simulink library "PacketizedNetworkLib"  (R2025b)
settings: Solver=VariableStepAuto  StartTime=0.0  StopTime=10.0  RelTol=1e-3
values from neighbouring files (symbols this model uses):
  dfeRef = [0.707106781187 -0.707106781187 0.707106781187 0.707106781187 -0.707106781187 0.707106781187 0.707106781187 0.707106781187 0.707106781187 0.707106781187 -0.707106781187 0.707106781187 ... (500 elements, 500x1)]    [networkParams.mat]
  L3payload = [0 0 0 1 0 0 0 0 1 1 1 0 ... (1040 elements, 1040x1)]    [networkParams.mat]
  ppdu_bb = [0 0 1 1 0 0 0 0 1 1 0 0 ... (2280 elements, 2280x1)]    [networkParams.mat]
  Ts = 1e-07    [networkParams.mat]
undefined symbols (not defined in the file or in its folder): AckDestAddre, DestAddre, dfilt, High, lambda, NodeAddre, pseed
libraries: $bdroot x19, hdlsllib x5, dspsigops x5, dspswit3 x3, simulink x3, dspindex x3, commdigbbndpm3 x2, simulink_extras x2, commfilt2 x2, commchan3 x1, dspmathops x1, dsparch4 x1
(part 1 of 3)
settings Model: Creator=The MathWorks, Inc.  LastModifiedBy=The MathWorks, Inc.
settings SolverCC: AlgebraicLoopSolver=TrustRegion
settings DataIOCC: ReturnWorkspaceOutputs=off
settings OptimizationCC: ReuseModelBlockBuffer=off
settings DebuggingCC: UnconnectedInputMsg=warning  UnconnectedOutputMsg=warning  UnconnectedLineMsg=warning  ArithmeticOperatorsInVariantConditions=warning
settings ModelReferenceCC: EnableRefExpFcnMdlSchedulingChecks=on
settings SFSimCC: SimUseLocalCustomCode=off  CustomCodeUndefinedFunction=UseInterfaceOnly
settings RTWCC: RTWUseLocalCustomCode=off  GPUComputeCapability=3.5

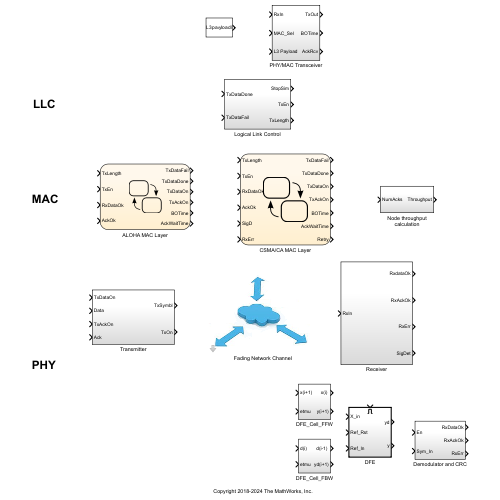
[thumbnail: Simulink's stored preview of the top-level diagram]
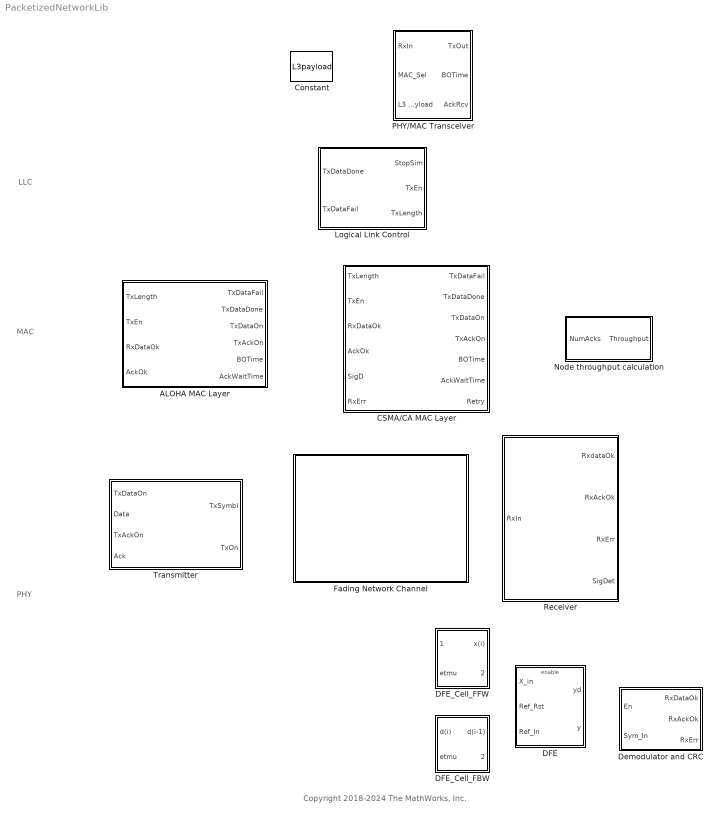
== system PacketizedNetworkLib ==
  note: PHY
  note: MAC
  note: LLC
  note: Copyright 2018-2024 The MathWorks, Inc.
  ALOHA MAC Layer : Stateflow chart  TreatAsAtomicUnit=on
  CSMA/CA MAC Layer : Stateflow chart  TreatAsAtomicUnit=on
  Constant : Constant  Value=L3payload
  DFE : Subsystem
  DFE_Cell_FBW : Subsystem
  DFE_Cell_FFW : Subsystem
  Demodulator and CRC : Subsystem
  Fading Network Channel : Subsystem  mask(Radio Network){MDSN12=0.000005/Ts, SNRN12=25, MDSN23=0.000005/Ts, SNRN23=25, MDSN31=0.000005/Ts, SNRN31=25}
      mask prompts: MDSN12 "Maximum Doppler Shift (Hz)"; SNRN12 "SNR of AWGN (Eb/No)"; MDSN23 "Maximum Doppler Shift (Hz)"; SNRN23 "SNR of AWGN (Eb/No)"; MDSN31 "Maximum Doppler Shift (Hz)"; SNRN31 "SNR of AWGN (Eb/No)"
      mask help: This model presents a radio network with Rayleigh fading channel between the transceiver nades.
      mask DialogControl ParameterGroupVar Prompt: Parameters for Channels
      mask DialogControl Container3 Prompt: Channel between Node 1 and Node 2
      mask DialogControl Container4 Prompt: Node 2 and Node 3
      mask DialogControl Container5 Prompt: Node 3 and Node 1
      mask Display: image('NetworkChannel.png');
  Logical Link Control : Subsystem
  Node throughput calculation : Subsystem
  PHY/MAC Transceiver : Subsystem
  Receiver : Subsystem
  Transmitter : Subsystem  Tag=safddsaf  Description=afsd as

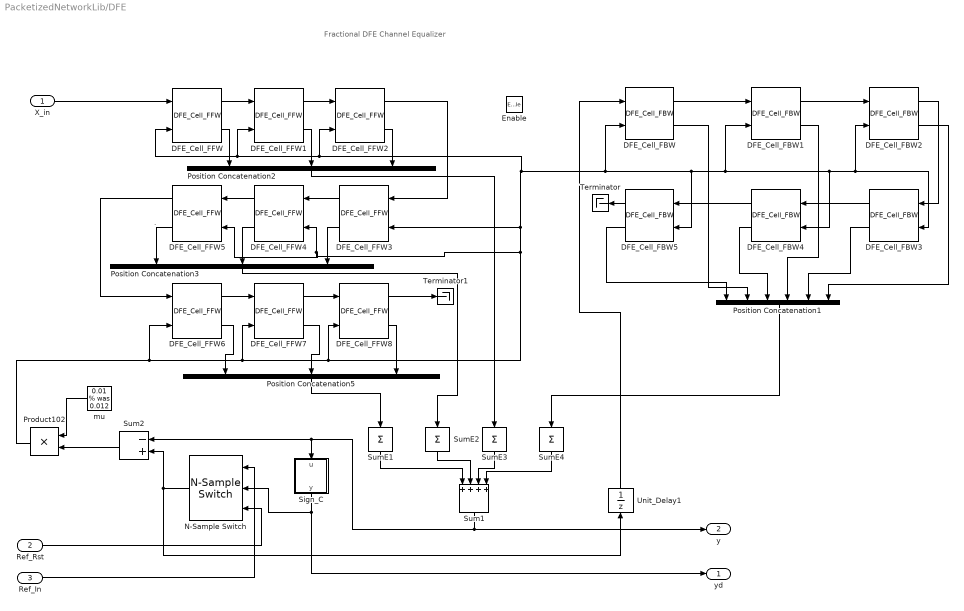
== system PacketizedNetworkLib/DFE ==
  note: .
  note: Fractional DFE Channel Equalizer
  X_in : Inport
  "Ref_Rst " : Inport  Port=2
  Ref_In : Inport  Port=3
  Enable : EnablePort
  DFE_Cell_FBW{,1..5} (6 alike) : $bdroot/DFE_Cell_FBW  SystemSampleTime=-1  VariantActivationTime=update diagram  EmptyChoice=off  PassThrough=off  PassThroughVariantControl=(default)  EmptyChoiceVariantControl=(default)  AllowFlexibleInterface=on  Latency=0  AutoFrameSizeCalculation=off
  DFE_Cell_FFW{,1..8} (9 alike) : $bdroot/DFE_Cell_FFW  SystemSampleTime=-1  VariantActivationTime=update diagram  EmptyChoice=off  PassThrough=off  PassThroughVariantControl=(default)  EmptyChoiceVariantControl=(default)  AllowFlexibleInterface=on  Latency=0  AutoFrameSizeCalculation=off
  N-Sample Switch : dspswit3/N-Sample Switch  N=152  reset=on  TriggerType=Rising edge  Ts=-1
  Position Concatenation1 : Concatenate  NumInputs=6  ConcatenateDimension=6
  Position Concatenation2 : Concatenate  NumInputs=3  ConcatenateDimension=3
  Position Concatenation3 : Concatenate  NumInputs=3  ConcatenateDimension=3
  Position Concatenation5 : Concatenate  NumInputs=3  ConcatenateDimension=3
  Product102 : Product  InputSameDT=on  RndMeth=Zero  SaturateOnIntegerOverflow=on  OutDataTypeStr=Inherit: Same as first input
  "Sign_C " : MATLAB Function  TreatAsAtomicUnit=on
  Sum1 : Sum  Inputs=++++  InputSameDT=on  SaturateOnIntegerOverflow=on  OutDataTypeStr=Inherit: Same as first input
  Sum2 : Sum  Inputs=-+  InputSameDT=on  SaturateOnIntegerOverflow=on  OutDataTypeStr=Inherit: Same as first input
  SumE{1..4} (4 alike) : Sum  Inputs=+
  Terminator : Terminator
  Terminator1 : Terminator
  "Unit_Delay1 " : UnitDelay  SampleTime=-1  HasFrameUpgradeWarning=on
  mu : Constant  Value="0.01  % was 0.012"  SampleTime=-1
  yd : Outport  VectorParamsAs1DForOutWhenUnconnected=off
  y : Outport  Port=2  VectorParamsAs1DForOutWhenUnconnected=off
  wires:
  DFE_Cell_FFW4/1 -> DFE_Cell_FFW5/1
  DFE_Cell_FFW3/2 -> Position Concatenation3/3
  Position Concatenation2/1 -> SumE3/1
  Position Concatenation3/1 -> SumE2/1
  DFE_Cell_FBW3/1 -> DFE_Cell_FBW4/1
  DFE_Cell_FFW7/2 -> Position Concatenation5/2
  DFE_Cell_FBW/1 -> DFE_Cell_FBW1/1
  DFE_Cell_FFW5/2 -> Position Concatenation3/1
  "Unit_Delay1 "/1 -> DFE_Cell_FBW/1
  DFE_Cell_FFW6/2 -> Position Concatenation5/1
  "Sign_C "/1(y) -> yd/1, N-Sample Switch/2
  DFE_Cell_FFW8/2 -> Position Concatenation5/3
  SumE2/1 -> Sum1/2
  DFE_Cell_FFW2/2 -> Position Concatenation2/3
  DFE_Cell_FFW8/1 -> Terminator1/1
  DFE_Cell_FFW5/1 -> DFE_Cell_FFW6/1
  Sum1/1 -> y/1, "Sign_C "/1(u), Sum2/1
  DFE_Cell_FFW1/2 -> Position Concatenation2/2
  DFE_Cell_FBW/2 -> Position Concatenation1/2
  DFE_Cell_FFW/2 -> Position Concatenation2/1
  SumE1/1 -> Sum1/1
  DFE_Cell_FFW3/1 -> DFE_Cell_FFW4/1
  DFE_Cell_FFW4/2 -> Position Concatenation3/2
  DFE_Cell_FBW5/1 -> Terminator/1
  Sum2/1 -> Product102/2
  DFE_Cell_FBW2/1 -> DFE_Cell_FBW3/1
  Product102/1 -> DFE_Cell_FFW6/2, DFE_Cell_FFW7/2, DFE_Cell_FFW8/2, DFE_Cell_FFW5/2, DFE_Cell_FFW4/2, DFE_Cell_FFW3/2, DFE_Cell_FFW2/2, DFE_Cell_FFW1/2, DFE_Cell_FFW/2, DFE_Cell_FBW/2, DFE_Cell_FBW5/2, DFE_Cell_FBW1/2, DFE_Cell_FBW4/2, DFE_Cell_FBW3/2, DFE_Cell_FBW2/2
  SumE3/1 -> Sum1/3
  mu/1 -> Product102/1
  N-Sample Switch/1 -> "Unit_Delay1 "/1, Sum2/2
  Position Concatenation1/1 -> SumE4/1
  DFE_Cell_FFW2/1 -> DFE_Cell_FFW3/1
  DFE_Cell_FFW1/1 -> DFE_Cell_FFW2/1
  DFE_Cell_FBW1/2 -> Position Concatenation1/4
  DFE_Cell_FBW3/2 -> Position Concatenation1/5
  DFE_Cell_FBW4/2 -> Position Concatenation1/3
  DFE_Cell_FBW4/1 -> DFE_Cell_FBW5/1
  DFE_Cell_FBW5/2 -> Position Concatenation1/1
  DFE_Cell_FBW1/1 -> DFE_Cell_FBW2/1
  SumE4/1 -> Sum1/4
  DFE_Cell_FFW/1 -> DFE_Cell_FFW1/1
  Position Concatenation5/1 -> SumE1/1
  DFE_Cell_FBW2/2 -> Position Concatenation1/6
  DFE_Cell_FFW6/1 -> DFE_Cell_FFW7/1
  DFE_Cell_FFW7/1 -> DFE_Cell_FFW8/1
  Ref_In/1 -> N-Sample Switch/1
  X_in/1 -> DFE_Cell_FFW/1
  "Ref_Rst "/1 -> N-Sample Switch/3

== system PacketizedNetworkLib/DFE_Cell_FBW ==
  note: w(i+1)
  note: The Basic Cell of the Feedbackward Part of DFE Equalizer
      |
      | yd(i+1)= w(i+1).*d(i);
      | w(i+1)=w(i)+ m*D* w(i)=w(i)+etmu*conj(x(i));
      |
      | Note: All variables here are scalars
  note: w(i)
  d(i) : Inport
  etmu : Inport  Port=2
  " Unit_Delay1" : UnitDelay  SampleTime=-1  HasFrameUpgradeWarning=on
  " Unit_Delay2" : UnitDelay  SampleTime=-1  HasFrameUpgradeWarning=on
  Math Function : Math  Operator=conj  SignedPower=on
  Product1 : Product  InputSameDT=on  RndMeth=Zero  SaturateOnIntegerOverflow=on  OutDataTypeStr=Inherit: Same as first input
  Product2 : Product  InputSameDT=on  RndMeth=Zero  SaturateOnIntegerOverflow=on  OutDataTypeStr=Inherit: Same as first input
  Sum : Sum  InputSameDT=on  SaturateOnIntegerOverflow=on  OutDataTypeStr=Inherit: Same as first input
  "Unit_Delay1 " : UnitDelay  SampleTime=-1  HasFrameUpgradeWarning=on
  "d(i-1) " : Outport  VectorParamsAs1DForOutWhenUnconnected=off
  yd(i+1) : Outport  Port=2  VectorParamsAs1DForOutWhenUnconnected=off
  wires:
  Product2/1 -> Sum/2
  Product1/1 -> yd(i+1)/1
  Sum/1 -> Product1/1, " Unit_Delay2"/1
  " Unit_Delay2"/1 -> Sum/1
  "Unit_Delay1 "/1 -> Math Function/1, "d(i-1) "/1
  etmu/1 -> " Unit_Delay1"/1
  d(i)/1 -> Product1/2, "Unit_Delay1 "/1
  Math Function/1 -> Product2/2
  " Unit_Delay1"/1 -> Product2/1

== system PacketizedNetworkLib/DFE_Cell_FFW ==
  note: w(i)
  note: The Basic Cell of the Feedforward Part of DFE Equalizer
      |
      | y(i+1)= ElimentSum (w(i+1).*x(i+1));
      | w(i+1)=w(i)+ m*D* w(i)=w(i)+etmu*conj(x(i));
      |
      | Note: y(+1) and etmu is a scalar, and x(i), w(i) are 2x1 vector. "2" is the decimation factor 2
  note: w(i+1)
  x(i+1) : Inport
  etmu : Inport  Port=2
  " Unit_Delay1" : UnitDelay  SampleTime=-1  HasFrameUpgradeWarning=on
  " Unit_Delay2" : UnitDelay  SampleTime=-1  HasFrameUpgradeWarning=on
  Math Function : Math  Operator=conj  SignedPower=on
  Product1 : Product  InputSameDT=on  RndMeth=Zero  SaturateOnIntegerOverflow=on  OutDataTypeStr=Inherit: Same as first input
  Product2 : Product  InputSameDT=on  RndMeth=Zero  SaturateOnIntegerOverflow=on  OutDataTypeStr=Inherit: Same as first input
  Sum : Sum  InputSameDT=on  SaturateOnIntegerOverflow=on  OutDataTypeStr=Inherit: Same as first input
  Sum of Elements : Sum  Inputs=+
  "Unit_Delay1 " : UnitDelay  SampleTime=-1  HasFrameUpgradeWarning=on
  "x(i) " : Outport  VectorParamsAs1DForOutWhenUnconnected=off
  y(i+1) : Outport  Port=2  VectorParamsAs1DForOutWhenUnconnected=off
  wires:
  " Unit_Delay1"/1 -> Product2/1
  Sum/1 -> " Unit_Delay2"/1, Product1/1
  Sum of Elements/1 -> y(i+1)/1
  Math Function/1 -> Product2/2
  x(i+1)/1 -> "Unit_Delay1 "/1, Product1/2
  etmu/1 -> " Unit_Delay1"/1
  "Unit_Delay1 "/1 -> "x(i) "/1, Math Function/1
  " Unit_Delay2"/1 -> Sum/1
  Product1/1 -> Sum of Elements/1
  Product2/1 -> Sum/2

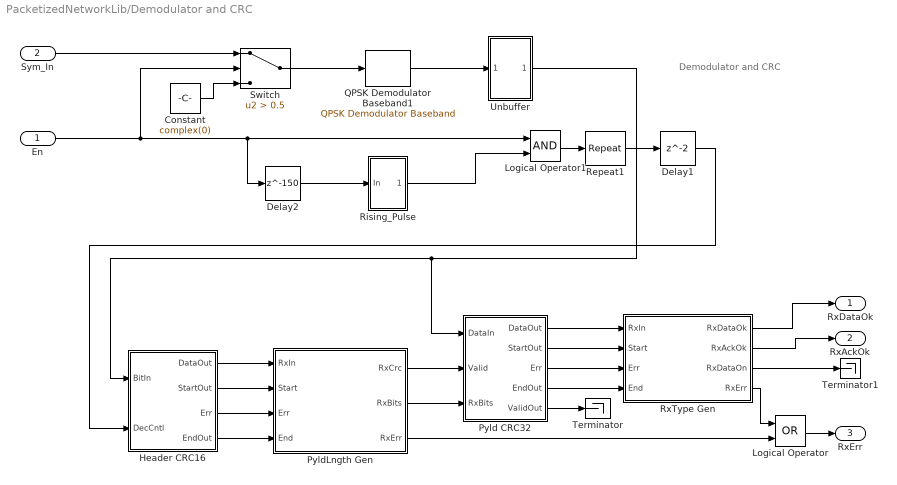
== system PacketizedNetworkLib/Demodulator and CRC ==
  note: Demodulator and CRC
  En : Inport
  Sym_In : Inport  Port=2
  " QPSK Demodulator Baseband1" : commdigbbndpm3/QPSK Demodulator Baseband  OutType=Bit  DecType=Hard decision  VarSource=Dialog  Variance=1  Dec=Gray  Ph=pi/4  outDtype1=Inherit via internal rule  outDtype2=Inherit via internal rule  derotateFactorWordLen=16  derotateFactorDataTypeStr=Inherit: Same word length as input  derotateFactorLastDataTypeStr=Inherit: Same word length as input
  Constant : Constant  Value=complex(0)  OutDataTypeStr=fixdt(1,16,14)  SampleTime=-1
  Delay1 : Delay
  Delay2 : Delay  DelayLength=150
  "Header CRC16 " : Subsystem
  Logical Operator : Logic  Operator=OR  AllPortsSameDT=off  OutDataTypeStr=boolean
  Logical Operator1 : Logic  AllPortsSameDT=off  OutDataTypeStr=boolean
  Pyld CRC32 : Subsystem
  PyldLngth Gen : Stateflow chart  TreatAsAtomicUnit=on
  Repeat1 : dspsigops/Repeat  FactorSource=Dialog parameter  N=2  Nmax=16  RateOptions=Allow multirate processing  ic=0  mode=Unused parameter value
  Rising_Pulse : Subsystem
  RxType Gen : Stateflow chart  TreatAsAtomicUnit=on
  Switch : Switch  Criteria=u2 > Threshold  Threshold=0.5  SaturateOnIntegerOverflow=off  InputSameDT=off
  Terminator : Terminator
  Terminator1 : Terminator
  Unbuffer : Subsystem
  RxDataOk : Outport  VectorParamsAs1DForOutWhenUnconnected=off
  RxAckOk : Outport  Port=2  VectorParamsAs1DForOutWhenUnconnected=off
  RxErr : Outport  Port=3  VectorParamsAs1DForOutWhenUnconnected=off
  wires:
  Pyld CRC32/1(DataOut) -> RxType Gen/1(RxIn)
  Switch/1 -> " QPSK Demodulator Baseband1"/1
  Constant/1 -> Switch/3
  Delay2/1 -> Rising_Pulse/1(In)
  Sym_In/1 -> Switch/1
  "Header CRC16 "/2(StartOut) -> PyldLngth Gen/2(Start)
  "Header CRC16 "/4(EndOut) -> PyldLngth Gen/4(End)
  "Header CRC16 "/3(Err) -> PyldLngth Gen/3(Err)
  PyldLngth Gen/1(RxCrc) -> Pyld CRC32/2(Valid)
  Rising_Pulse/1(Out1) -> Logical Operator1/2
  Unbuffer/1(Out1) -> Pyld CRC32/1(DataIn), "Header CRC16 "/1(BitIn)
  Pyld CRC32/2(StartOut) -> RxType Gen/2(Start)
  Pyld CRC32/3(Err) -> RxType Gen/3(Err)
  Pyld CRC32/4(EndOut) -> RxType Gen/4(End)
  RxType Gen/1(RxDataOk) -> RxDataOk/1
  RxType Gen/2(RxAckOk) -> RxAckOk/1
  En/1 -> Switch/2, Logical Operator1/1, Delay2/1
  " QPSK Demodulator Baseband1"/1 -> Unbuffer/1(In1)
  "Header CRC16 "/1(DataOut) -> PyldLngth Gen/1(RxIn)
  Pyld CRC32/5(ValidOut) -> Terminator/1
  PyldLngth Gen/3(RxErr) -> Logical Operator/2
  RxType Gen/4(RxErr) -> Logical Operator/1
  Logical Operator/1 -> RxErr/1
  Logical Operator1/1 -> Repeat1/1
  RxType Gen/3(RxDataOn) -> Terminator1/1
  PyldLngth Gen/2(RxBits) -> Pyld CRC32/3(RxBits)
  Repeat1/1 -> Delay1/1
  Delay1/1 -> "Header CRC16 "/2(DecCntl)

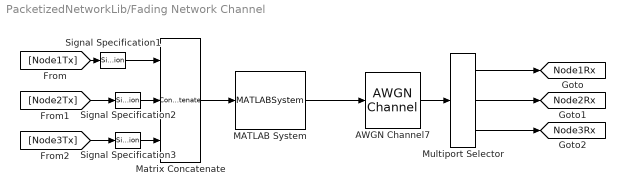
== system PacketizedNetworkLib/Fading Network Channel ==
  AWGN Channel7 : commchan3/AWGN Channel  LegacyMode=off  NoiseMethod="Signal to noise ratio  (Eb/No)"  noiseMode="Signal to noise ratio  (SNR)"  EbNo=[SNRN12, SNRN23, SNRN31]  EsNo=10  SNR=10  BitsPerSymbol=2  SignalPower=0.1634  SpecifySymbolPeriod=off  SamplesPerSymbol=1  SymbolPeriod=Ts  VarianceSource=Parameter  Variance=1  RandomStream=mt19937ar with seed  Seed=67  SimulateUsing=Code generation
  MATLAB System : MATLABSystem  System=NetworkChannel  SampleRateSource=Input port  SampleRate=[ 1e3, 2e3, 3e3 ]  PathDelays={[0 0.3*Ts], [0 0.3*Ts]; [0 0.3*Ts], [0 0.3*Ts]; [0 0.3*Ts], [0 0.3*Ts]}  AveragePathGains={[0 -6],[0 -6]; [0 -6],[0 -6]; [0 -6],[0 -6]}  MaximumDopplerShift=[MDSN12, MDSN31; MDSN23, MDSN12; MDSN31, MDSN23]  SimulateUsing=Code generation
      mask Type: NetworkChannel
  Matrix Concatenate : Concatenate  NumInputs=3  Mode=Multidimensional array  ConcatenateDimension=2
  Multiport Selector : dspindex/Multiport Selector  rowsOrCols=Columns  idxCellArray=num2cell(1:3)  idxErrMode=Clip Index
  Signal Specification1 : SignalSpecification  Dimensions=1
  Signal Specification2 : SignalSpecification  Dimensions=1
  Signal Specification3 : SignalSpecification  Dimensions=1
  tag scope: Node1Rx=global, Node2Rx=global, Node3Rx=global
  wires:
  [Node1Tx] -> Signal Specification1/1
  [Node2Tx] -> Signal Specification2/1
  [Node3Tx] -> Signal Specification3/1
  Matrix Concatenate/1 -> MATLAB System/1
  Signal Specification1/1 -> Matrix Concatenate/1
  Signal Specification2/1 -> Matrix Concatenate/2
  Signal Specification3/1 -> Matrix Concatenate/3
  Multiport Selector/1 -> [Node1Rx]
  Multiport Selector/2 -> [Node2Rx]
  Multiport Selector/3 -> [Node3Rx]
  AWGN Channel7/1 -> Multiport Selector/1
  MATLAB System/1 -> AWGN Channel7/1

== system PacketizedNetworkLib/Logical Link Control ==
  TxDataDone : Inport
  TxDataFail : Inport  Port=2
  Exponential Random Variable : Subsystem
  Logical Link Control : Stateflow chart  TreatAsAtomicUnit=on
  Terminator : Terminator
  Terminator1 : Terminator
  StopSim : Outport  VectorParamsAs1DForOutWhenUnconnected=off
  TxEn : Outport  Port=2  VectorParamsAs1DForOutWhenUnconnected=off
  TxLength : Outport  Port=3  VectorParamsAs1DForOutWhenUnconnected=off
  wires:
  Logical Link Control/2(TxEn) -> TxEn/1
  TxDataDone/1 -> Logical Link Control/1(TxDataDone)
  Logical Link Control/1(StopSim) -> StopSim/1
  Logical Link Control/5(TxMore) -> Terminator1/1
  TxDataFail/1 -> Logical Link Control/2(TxDataFail)
  Logical Link Control/4(TxWaitTime) -> Terminator/1
  Logical Link Control/3(TxLength) -> TxLength/1
  Exponential Random Variable/1(Out1) -> Logical Link Control/3(TxWaitUnits)

== system PacketizedNetworkLib/Node throughput calculation ==
  NumAcks : Inport
  Clock : Clock
  Cumulative Sum2 : dspmathops/Cumulative Sum  dim=Channels (running sum)  InputProcessing=Columns as channels (frame based)  reset_popup=None  roundingMode=Floor  overflowMode=off  outputDataTypeStr=Inherit: Same as accumulator  outputMin=[]  outputMax=[]  outputLastDataTypeStr=Inherit: Same as accumulator
  Data Type Conversion2 : DataTypeConversion  OutDataTypeStr=uint8  SaturateOnIntegerOverflow=off  RndMeth=Floor
  Data packet airtime : Constant  Value=(50+254+16+16+4+2+2+8+8+8+32+1040+32)/20e6
  Divide2 : Product  Inputs=*/
  Product2 : Product
  Throughput : Outport  VectorParamsAs1DForOutWhenUnconnected=off
  wires:
  Data packet airtime/1 -> Product2/2
  Cumulative Sum2/1 -> Product2/1
  Data Type Conversion2/1 -> Cumulative Sum2/1
  Product2/1 -> Divide2/1
  Divide2/1 -> Throughput/1
  Clock/1 -> Divide2/2
  NumAcks/1 -> Data Type Conversion2/1

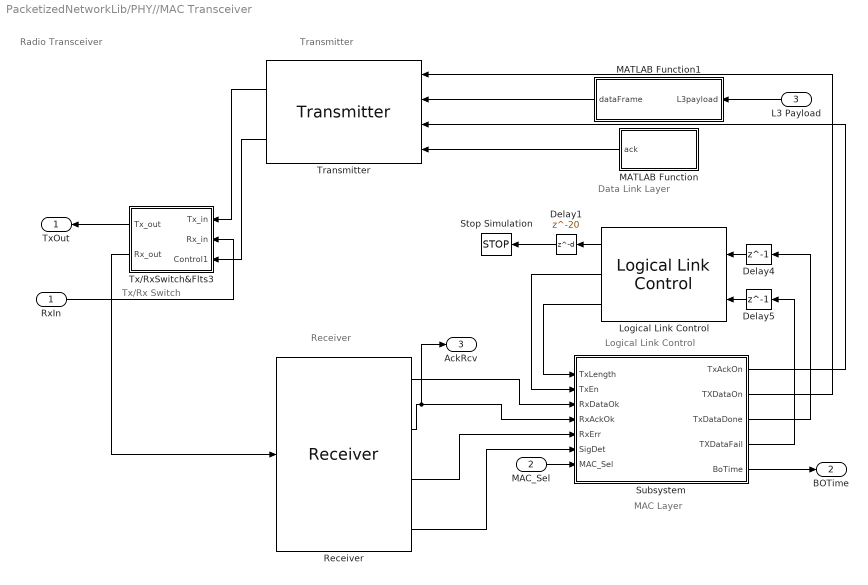
== system PacketizedNetworkLib/PHY//MAC Transceiver ==
  note: Data Link Layer
  note: Radio Transceiver
  note: Transmitter
  note: Receiver
  note: Tx/Rx Switch
  note: MAC Layer
  note: Logical Link Control
  RxIn : Inport
  MAC_Sel : Inport  Port=2
  L3 Payload : Inport  Port=3
  Delay1 : Delay  DelayLength=20  InitialCondition=0  UseCircularBuffer=on
  Delay4 : Delay  DelayLength=1  InitialCondition=0  UseCircularBuffer=on
  Delay5 : Delay  DelayLength=1  InitialCondition=0  UseCircularBuffer=on
  Logical Link Control : $bdroot/Logical Link Control  SystemSampleTime=-1  VariantActivationTime=update diagram  EmptyChoice=off  PassThrough=off  PassThroughVariantControl=(default)  EmptyChoiceVariantControl=(default)  AllowFlexibleInterface=on  Latency=0  AutoFrameSizeCalculation=off
  MATLAB Function : MATLAB Function  TreatAsAtomicUnit=on
  MATLAB Function1 : MATLAB Function  TreatAsAtomicUnit=on
  Receiver : $bdroot/Receiver  SystemSampleTime=-1  VariantActivationTime=update diagram  EmptyChoice=off  PassThrough=off  PassThroughVariantControl=(default)  EmptyChoiceVariantControl=(default)  AllowFlexibleInterface=on  Latency=0  AutoFrameSizeCalculation=off
  Stop Simulation : Stop
  Subsystem : Subsystem
  Transmitter : $bdroot/Transmitter  Tag=safddsaf  Description=afsd as  SystemSampleTime=-1  VariantActivationTime=update diagram  EmptyChoice=off  PassThrough=off  PassThroughVariantControl=(default)  EmptyChoiceVariantControl=(default)  AllowFlexibleInterface=on  Latency=0  AutoFrameSizeCalculation=off
  Tx/RxSwitch&Flts3 : Subsystem
  TxOut : Outport  VectorParamsAs1DForOutWhenUnconnected=off
  BOTime : Outport  Port=2  VectorParamsAs1DForOutWhenUnconnected=off
  AckRcv : Outport  Port=3  VectorParamsAs1DForOutWhenUnconnected=off
  wires:
  Tx/RxSwitch&Flts3/2(Rx_out) -> Receiver/1
  Delay4/1 -> Logical Link Control/1
  Tx/RxSwitch&Flts3/1(Tx_out) -> TxOut/1
  Delay5/1 -> Logical Link Control/2
  Delay1/1 -> Stop Simulation/1
  Logical Link Control/1 -> Delay1/1
  Transmitter/2 -> Tx/RxSwitch&Flts3/3(Control1)
  RxIn/1 -> Tx/RxSwitch&Flts3/2(Rx_in)
  Transmitter/1 -> Tx/RxSwitch&Flts3/1(Tx_in)
  Receiver/1 -> Subsystem/3(RxDataOk)
  Logical Link Control/2 -> Subsystem/2(TxEn)
  Logical Link Control/3 -> Subsystem/1(TxLength)
  Receiver/2 -> AckRcv/1, Subsystem/4(RxAckOk)
  Subsystem/1(TxAckOn) -> Transmitter/3
  Subsystem/2(TXDataOn) -> Transmitter/1
  Subsystem/3(TxDataDone) -> Delay4/1
  Subsystem/4(TXDataFail) -> Delay5/1
  Receiver/3 -> Subsystem/5(RxErr)
  MAC_Sel/1 -> Subsystem/7(MAC_Sel)
  Subsystem/5(BoTime) -> BOTime/1
  MATLAB Function/1(ack) -> Transmitter/4
  L3 Payload/1 -> MATLAB Function1/1(L3payload)
  MATLAB Function1/1(dataFrame) -> Transmitter/2
  Receiver/4 -> Subsystem/6(SigDet)

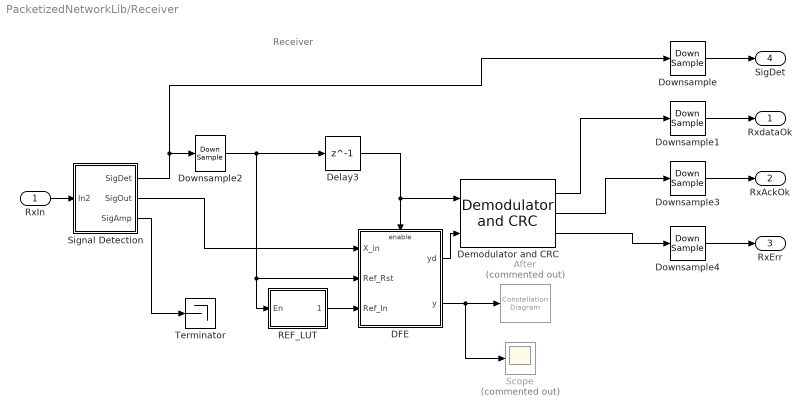
== system PacketizedNetworkLib/Receiver ==
  note: Receiver
  RxIn : Inport
  After : ConstellationDiagram  Tag=ScatterPlot  Commented=on  WindowPosition=[1082 641 454 346]  SymbolsToDisplaySource=Property  SymbolsToDisplay=800  Title=Scatter Plot  XLimits=[-1 1]  YLimits=[-1 1]  AxesLimits=[-1 1]  ShowReferenceConstellation=off  ColorFading=on  DefaultConfigurationName=comm.scopes.ConstellationDiagramBlockCfg
  "DFE " : Subsystem
  Delay3 : Delay  DelayLength=1
  Demodulator and CRC : $bdroot/Demodulator and CRC  SystemSampleTime=-1  VariantActivationTime=update diagram  EmptyChoice=off  PassThrough=off  PassThroughVariantControl=(default)  EmptyChoiceVariantControl=(default)  AllowFlexibleInterface=on  Latency=0  AutoFrameSizeCalculation=off
  Downsample{,1,3..4} (4 alike) : DownSample  N=16  RateOptions=Allow multirate processing
  Downsample2 : DownSample  RateOptions=Allow multirate processing
  REF_LUT : Subsystem
  Scope : Scope  Commented=on
      settings: ActiveDisplayYMinimum=-1.43192  ActiveDisplayYMaximum=1.60722  DataLoggingVariableName=ScopeData4  DataLoggingSaveFormat=Array
  Signal Detection : Subsystem
  Terminator : Terminator
  RxdataOk : Outport  VectorParamsAs1DForOutWhenUnconnected=off
  RxAckOk : Outport  Port=2  VectorParamsAs1DForOutWhenUnconnected=off
  RxErr : Outport  Port=3  VectorParamsAs1DForOutWhenUnconnected=off
  SigDet : Outport  Port=4  VectorParamsAs1DForOutWhenUnconnected=off
  wires:
  Downsample/1 -> SigDet/1
  Signal Detection/3(SigAmp) -> Terminator/1
  Downsample2/1 -> Delay3/1, REF_LUT/1(En), "DFE "/2("Ref_Rst ")
  Delay3/1 -> Demodulator and CRC/1, "DFE "/Enable
  Demodulator and CRC/2 -> Downsample3/1
  Signal Detection/2(SigOut) -> "DFE "/1(X_in)
  REF_LUT/1(DataOut) -> "DFE "/3(Ref_In)
  Signal Detection/1(SigDet) -> Downsample/1, Downsample2/1
  "DFE "/1(yd) -> Demodulator and CRC/2
  RxIn/1 -> Signal Detection/1(In2)
  "DFE "/2(y) -> Scope/1, After/1
  Demodulator and CRC/3 -> Downsample4/1
  Downsample1/1 -> RxdataOk/1
  Demodulator and CRC/1 -> Downsample1/1
  Downsample3/1 -> RxAckOk/1
  Downsample4/1 -> RxErr/1

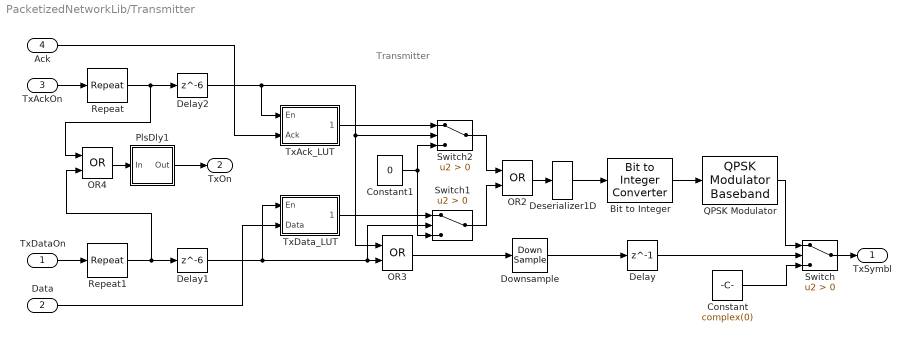
== system PacketizedNetworkLib/Transmitter ==
  note: Transmitter
  TxDataOn : Inport
  Data : Inport  Port=2
  TxAckOn : Inport  Port=3
  Ack : Inport  Port=4
  Bit to Integer : simulink/Logic and Bit Operations/Bit to Integer Converter  nbits=2  bitOrder=LSB first  signedOutputValues=Unsigned  outDtype=Inherit via internal rule  outDtypeSigned=Inherit via internal rule
      settings: LibrarySourceBlock=|
      | commutil2/Bit to Integer
      | Converter
  Constant : Constant  Value=complex(0)
  Constant1 : Constant  Value=0
  Delay : Delay  DelayLength=1
  Delay1 : Delay  DelayLength=6
  Delay2 : Delay  DelayLength=6
  Deserializer1D : hdlsllib/HDL Operations/Deserializer1D  Ratio=2  IdleCycles=0  InitialCondition=0  startIn=off  validIn=off  validOut=off  inputDataDimensions=-1  inputSampleTime=-1  inputSignalType=auto
  Downsample : DownSample  RateOptions=Allow multirate processing
  OR2 : Logic  Operator=OR  AllPortsSameDT=off  OutDataTypeStr=boolean
  OR3 : Logic  Operator=OR  AllPortsSameDT=off  OutDataTypeStr=boolean
  OR4 : Logic  Operator=OR  AllPortsSameDT=off  OutDataTypeStr=boolean
  PlsDly1 : Subsystem
  QPSK Modulator : commdigbbndpm3/QPSK Modulator Baseband  InType=Integer  Enc=Gray  Ph=pi/4  outDtype=double  outWordLen=16  outUDDataType=sfix(16)  outFracLenMode=Best precision  outFracLen=15  outDataTypeStr=double  outLastDataTypeStr=double
  Repeat : dspsigops/Repeat  FactorSource=Dialog parameter  N=16  Nmax=16  InputProcessing=Columns as channels (frame based)  RateOptions=Allow multirate processing  ic=0  mode=Unused parameter value
  Repeat1 : dspsigops/Repeat  FactorSource=Dialog parameter  N=16  Nmax=16  InputProcessing=Columns as channels (frame based)  RateOptions=Allow multirate processing  ic=0  mode=Unused parameter value
  Switch : Switch  Criteria=u2 > Threshold  SaturateOnIntegerOverflow=off  InputSameDT=off
  Switch1 : Switch  Criteria=u2 > Threshold  SaturateOnIntegerOverflow=off  InputSameDT=off
  Switch2 : Switch  Criteria=u2 > Threshold  SaturateOnIntegerOverflow=off  InputSameDT=off
  TxAck_LUT : Subsystem
  TxData_LUT : Subsystem
  TxSymbl : Outport  VectorParamsAs1DForOutWhenUnconnected=off
  TxOn : Outport  Port=2  VectorParamsAs1DForOutWhenUnconnected=off
  wires:
  TxData_LUT/1(DataOut) -> Switch1/1
  PlsDly1/1(Out) -> TxOn/1
  Repeat1/1 -> OR4/2, Delay1/1
  TxDataOn/1 -> Repeat1/1
  Repeat/1 -> OR4/1, Delay2/1
  TxAckOn/1 -> Repeat/1
  Deserializer1D/1 -> Bit to Integer/1
  Switch/1 -> TxSymbl/1
  QPSK Modulator/1 -> Switch/1
  Switch2/1 -> OR2/1
  Switch1/1 -> OR2/2
  TxAck_LUT/1(DataOut) -> Switch2/1
  Delay/1 -> Switch/2
  Downsample/1 -> Delay/1
  Constant/1 -> Switch/3
  OR2/1 -> Deserializer1D/1
  OR3/1 -> Downsample/1
  Constant1/1 -> Switch1/3, Switch2/3
  Bit to Integer/1 -> QPSK Modulator/1
  Delay1/1 -> Switch1/2, OR3/2, TxData_LUT/1(En)
  Delay2/1 -> OR3/1, Switch2/2, TxAck_LUT/1(En)
  OR4/1 -> PlsDly1/1(In)
  Ack/1 -> TxAck_LUT/2(Ack)
  Data/1 -> TxData_LUT/2(Data)

== system PacketizedNetworkLib/Demodulator and CRC/Header CRC16  ==
  BitIn : Inport
  DecCntl : Inport  Port=2
  CRC_Check16W : Subsystem
  Data Type Conversion : DataTypeConversion  OutDataTypeStr=boolean  SaturateOnIntegerOverflow=off  RndMeth=Floor
  Data Type2 : DataTypeConversion  OutDataTypeStr=boolean  SaturateOnIntegerOverflow=off  RndMeth=Floor
  Terminator : Terminator
  DataOut : Outport  VectorParamsAs1DForOutWhenUnconnected=off
  StartOut : Outport  Port=2  VectorParamsAs1DForOutWhenUnconnected=off
  Err : Outport  Port=3  VectorParamsAs1DForOutWhenUnconnected=off
  EndOut : Outport  Port=4  VectorParamsAs1DForOutWhenUnconnected=off
  wires:
  CRC_Check16W/5(ValidOut) -> Terminator/1
  CRC_Check16W/4(EndOut) -> EndOut/1
  CRC_Check16W/1(DataOut) -> DataOut/1
  CRC_Check16W/2(StartOut) -> StartOut/1
  CRC_Check16W/3(Err) -> Err/1
  Data Type2/1 -> CRC_Check16W/1(DataIn)
  Data Type Conversion/1 -> CRC_Check16W/2(Valid)
  BitIn/1 -> Data Type2/1
  DecCntl/1 -> Data Type Conversion/1

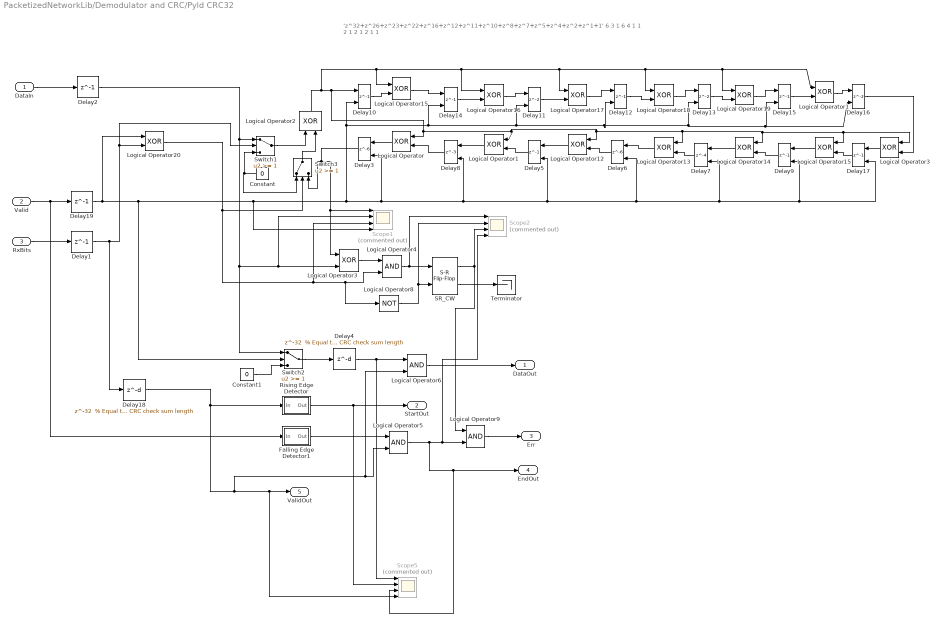
== system PacketizedNetworkLib/Demodulator and CRC/Pyld CRC32 ==
  note: 'z^32+z^26+z^23+z^22+z^16+z^12+z^11+z^10+z^8+z^7+z^5+z^4+z^2+z^1+1'
      | 6 3 1 6 4 1 1 2 1 2 1 2 1 1
  DataIn : Inport
  Valid : Inport  Port=2
  RxBits : Inport  Port=3
  Constant : Constant  Value=0  OutDataTypeStr=boolean  SampleTime=-1
  Constant1 : Constant  Value=0  OutDataTypeStr=boolean  SampleTime=-1
  Delay1 : Delay  DelayLength=1
  Delay{5,9..10,12,14..15,17} (7 alike) : Delay  DelayLength=1  InitialCondition=0  ExternalReset=Rising
      settings: InputPortMap=u0,r5
  Delay11 : Delay  InitialCondition=0  ExternalReset=Rising
      settings: InputPortMap=u0,r5
  Delay13 : Delay  InitialCondition=0  ExternalReset=Rising
      settings: InputPortMap=u0,r5
  Delay16 : Delay  InitialCondition=0  ExternalReset=Rising
      settings: InputPortMap=u0,r5
  Delay18 : Delay  DelayLength="32  % Equal to the CRC check sum length"  InitialCondition=0
  Delay19 : Delay  DelayLength=1
  Delay2 : Delay  DelayLength=1
  Delay3 : Delay  DelayLength=6  InitialCondition=0  ExternalReset=Rising
      settings: InputPortMap=u0,r5
  Delay4 : Delay  DelayLength="32  % Equal to the CRC check sum length"  InitialCondition=0
  Delay6 : Delay  DelayLength=6  InitialCondition=0  ExternalReset=Rising
      settings: InputPortMap=u0,r5
  Delay7 : Delay  DelayLength=4  InitialCondition=0  ExternalReset=Rising
      settings: InputPortMap=u0,r5
  Delay8 : Delay  DelayLength=3  InitialCondition=0  ExternalReset=Rising
      settings: InputPortMap=u0,r5
  Falling Edge Detector1 : Subsystem
  Logical Operator{,1,1..3,3,12..15,15..20} (16 alike) : Logic  Operator=XOR  AllPortsSameDT=off  OutDataTypeStr=boolean
  Logical Operator{4..6,9} (4 alike) : Logic  AllPortsSameDT=off  OutDataTypeStr=boolean
  Logical Operator8 : Logic  Operator=NOT  AllPortsSameDT=off  OutDataTypeStr=boolean
  Rising Edge Detector : Subsystem
  SR_CW : simulink_extras/Flip Flops/S-R Flip-Flop  initial_condition=0
  Scope1 : Scope  Commented=on  NumInputPorts=4
      settings: ActiveDisplayYMinimum=-0.125  ActiveDisplayYMaximum=1.125  DataLoggingVariableName=ScopeData4  DataLoggingSaveFormat=Array
  Scope2 : Scope  Commented=on  NumInputPorts=4
      settings: ActiveDisplayYMinimum=-0.125  ActiveDisplayYMaximum=1.125  DataLoggingSaveFormat=Array
  Scope5 : Scope  Commented=on  NumInputPorts=4
      settings: ActiveDisplayYMinimum=-0.125  ActiveDisplayYMaximum=1.125  DataLoggingVariableName=ScopeData2  DataLoggingSaveFormat=Array
  Switch1 : Switch  Threshold=1  OutDataTypeStr=Inherit: Inherit via back propagation  SaturateOnIntegerOverflow=off
  Switch2 : Switch  Threshold=1  OutDataTypeStr=Inherit: Inherit via back propagation  SaturateOnIntegerOverflow=off
  Switch3 : Switch  Threshold=1  OutDataTypeStr=Inherit: Inherit via back propagation  SaturateOnIntegerOverflow=off
  Terminator : Terminator
  DataOut : Outport  VectorParamsAs1DForOutWhenUnconnected=off
  StartOut : Outport  Port=2  VectorParamsAs1DForOutWhenUnconnected=off
  Err : Outport  Port=3  VectorParamsAs1DForOutWhenUnconnected=off
  EndOut : Outport  Port=4  VectorParamsAs1DForOutWhenUnconnected=off
  ValidOut : Outport  Port=5  VectorParamsAs1DForOutWhenUnconnected=off
  wires:
  Logical Operator6/1 -> DataOut/1
  Logical Operator5/1 -> Logical Operator9/2, Scope2/4, EndOut/1, Scope5/3
  Delay18/1 -> Rising Edge Detector/1(In), ValidOut/1, Scope5/4, Logical Operator5/2, Logical Operator6/2
  Delay1/1 -> Delay18/1, Switch1/2, Logical Operator20/2
  Delay3/1 -> Switch3/3, Logical Operator3/1, Scope1/1
  Logical Operator20/1 -> Switch3/2, Scope1/3, Logical Operator8/1, Logical Operator4/2
  Switch1/1 -> Logical Operator2/1
  Constant/1 -> Switch3/1, Switch1/3
  Switch3/1 -> Logical Operator2/2
  RxBits/1 -> Delay1/1
  Delay19/1 -> Switch2/2, Delay17/2, Delay9/2, Delay7/2, Delay6/2, Delay5/2, Delay8/2, Delay3/2, Delay10/2, Delay14/2, Delay11/2, Delay13/2, Delay16/2, Delay15/2, Delay12/2, Scope1/4, Logical Operator20/1
  Delay16/1 -> Logical Operator3/2
  Logical Operator1/1 -> Delay16/1
  Delay15/1 -> Logical Operator1/2
  Logical Operator19/1 -> Delay15/1
  Delay13/1 -> Logical Operator19/2
  Logical Operator18/1 -> Delay13/1
  Delay12/1 -> Logical Operator18/2
  Logical Operator17/1 -> Delay12/1
  Delay11/1 -> Logical Operator17/2
  Logical Operator16/1 -> Delay11/1
  Delay14/1 -> Logical Operator16/2
  Logical Operator15/1 -> Delay14/1
  Delay10/1 -> Logical Operator15/2
  Delay17/1 -> Logical Operator15/2
  Delay9/1 -> Logical Operator14/2
  Delay7/1 -> Logical Operator13/2
  Delay6/1 -> Logical Operator12/2
  Delay5/1 -> Logical Operator1/2
  Delay8/1 -> Logical Operator/2
  Logical Operator3/1 -> Delay17/1
  Logical Operator15/1 -> Delay9/1
  Logical Operator14/1 -> Delay7/1
  Logical Operator13/1 -> Delay6/1
  Logical Operator12/1 -> Delay5/1
  Logical Operator/1 -> Delay3/1
  Falling Edge Detector1/1(Out) -> Logical Operator5/1
  Switch2/1 -> Delay4/1
  Constant1/1 -> Switch2/3
  Valid/1 -> Delay19/1, Falling Edge Detector1/1(In)
  Logical Operator1/1 -> Delay8/1
  Logical Operator8/1 -> Scope2/2, SR_CW/2
  Logical Operator3/1 -> Logical Operator4/1
  Logical Operator4/1 -> Scope2/1, SR_CW/1
  DataIn/1 -> Delay2/1
  Delay2/1 -> Logical Operator3/2, Scope1/2, Switch2/1, Switch1/1
  Logical Operator9/1 -> Err/1
  SR_CW/1 -> Scope2/3, Logical Operator9/1
  Delay4/1 -> Scope5/1, Logical Operator6/1
  Rising Edge Detector/1(Out) -> StartOut/1, Scope5/2
  SR_CW/2 -> Terminator/1
  Logical Operator2/1 -> Delay10/1, Logical Operator/1, Logical Operator1/1, Logical Operator12/1, Logical Operator13/1, Logical Operator14/1, Logical Operator15/1, Logical Operator3/1, Logical Operator16/1, Logical Operator17/1, Logical Operator1/1, Logical Operator19/1, Logical Operator18/1, Logical Operator15/1

== system PacketizedNetworkLib/Demodulator and CRC/Rising_Pulse ==
  In : Inport
  Delay : Delay  DelayLength=16  ExternalReset=Rising
      settings: InputPortMap=u0,r5
  Logical Operator : Logic  AllPortsSameDT=off  OutDataTypeStr=boolean
  Logical Operator2 : Logic  Operator=NOT  AllPortsSameDT=off  OutDataTypeStr=boolean
  Out1 : Outport  VectorParamsAs1DForOutWhenUnconnected=off
  wires:
  Logical Operator/1 -> Out1/1
  Delay/1 -> Logical Operator2/1
  Logical Operator2/1 -> Logical Operator/2
  In/1 -> Delay/2, Delay/1, Logical Operator/1

== system PacketizedNetworkLib/Demodulator and CRC/Unbuffer ==
  In1 : Inport
  Delay : Delay  DelayLength=1  InitialCondition=0  UseCircularBuffer=on
  Demux : Demux  Outputs=2
  Logical Operator : Logic  Operator=OR  AllPortsSameDT=off  OutDataTypeStr=boolean
  Upsample : dspsigops/Upsample  FactorSource=Dialog parameter  N=2  Nmax=16  phase=0  RateOptions=Allow multirate processing  ic=0  mode=Unused parameter value
  Upsample1 : dspsigops/Upsample  FactorSource=Dialog parameter  N=2  Nmax=16  phase=0  RateOptions=Allow multirate processing  ic=0  mode=Unused parameter value
  Out1 : Outport  VectorParamsAs1DForOutWhenUnconnected=off
  wires:
  In1/1 -> Demux/1
  Demux/2 -> Upsample/1
  Demux/1 -> Upsample1/1
  Upsample1/1 -> Delay/1
  Delay/1 -> Logical Operator/1
  Upsample/1 -> Logical Operator/2
  Logical Operator/1 -> Out1/1

== system PacketizedNetworkLib/Logical Link Control/Exponential Random Variable ==
  note: Inverse Transform Method:
      | Generate an exponential random variable from a uniform random variable
  Gain : Gain  Gain=-1/lambda
  Math Function : Math  Operator=log  SignedPower=on
  Uniform Random Number : UniformRandomNumber  Minimum=0  Seed=pseed  SampleTime=8e-7
  Out1 : Outport  VectorParamsAs1DForOutWhenUnconnected=off
  wires:
  Math Function/1 -> Gain/1
  Uniform Random Number/1 -> Math Function/1
  Gain/1 -> Out1/1

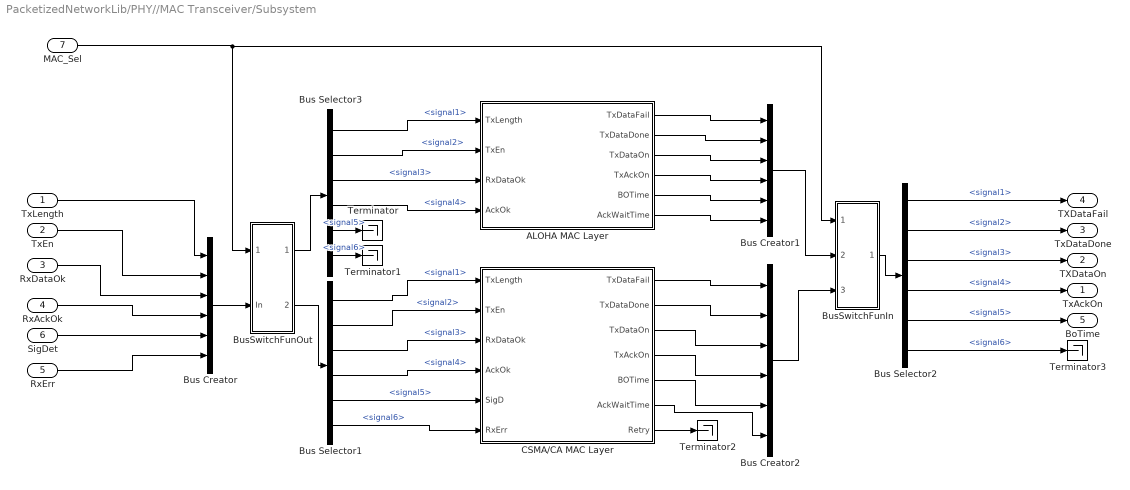
== system PacketizedNetworkLib/PHY//MAC Transceiver/Subsystem ==
  TxLength : Inport
  TxEn : Inport  Port=2
  RxDataOk : Inport  Port=3
  RxAckOk : Inport  Port=4
  RxErr : Inport  Port=5
  SigDet : Inport  Port=6
  MAC_Sel : Inport  Port=7
  ALOHA MAC Layer : Stateflow chart  TreatAsAtomicUnit=on
  Bus Creator : BusCreator  Inputs=6
  Bus Creator1 : BusCreator  Inputs=6
  Bus Creator2 : BusCreator  Inputs=6
  Bus Selector1 : BusSelector  OutputSignals=signal1,signal2,signal3,signal4,signal5,signal6
  Bus Selector2 : BusSelector  OutputSignals=signal1,signal2,signal3,signal4,signal5,signal6
  Bus Selector3 : BusSelector  OutputSignals=signal1,signal2,signal3,signal4,signal5,signal6
  BusSwitchFunIn : Subsystem
  BusSwitchFunOut : Subsystem
  CSMA/CA MAC Layer : Stateflow chart  TreatAsAtomicUnit=on
  Terminator{,1..3} (4 alike) : Terminator
  TxAckOn : Outport  VectorParamsAs1DForOutWhenUnconnected=off
  TXDataOn : Outport  Port=2  VectorParamsAs1DForOutWhenUnconnected=off
  TxDataDone : Outport  Port=3  VectorParamsAs1DForOutWhenUnconnected=off
  TXDataFail : Outport  Port=4  VectorParamsAs1DForOutWhenUnconnected=off
  BoTime : Outport  Port=5  VectorParamsAs1DForOutWhenUnconnected=off
  wires:
  Bus Selector3/2 -> ALOHA MAC Layer/2(TxEn)  "<signal2>"
  Bus Selector1/1 -> CSMA/CA MAC Layer/1(TxLength)  "<signal1>"
  Bus Selector3/1 -> ALOHA MAC Layer/1(TxLength)  "<signal1>"
  RxAckOk/1 -> Bus Creator/4
  Bus Selector3/4 -> ALOHA MAC Layer/4(AckOk)  "<signal4>"
  Bus Selector1/4 -> CSMA/CA MAC Layer/4(AckOk)  "<signal4>"
  Bus Selector1/2 -> CSMA/CA MAC Layer/2(TxEn)  "<signal2>"
  Bus Selector3/3 -> ALOHA MAC Layer/3(RxDataOk)  "<signal3>"
  RxErr/1 -> Bus Creator/6
  BusSwitchFunOut/2(Out2) -> Bus Selector1/1
  Bus Selector1/3 -> CSMA/CA MAC Layer/3(RxDataOk)  "<signal3>"
  Bus Creator/1 -> BusSwitchFunOut/2(In)
  Bus Selector1/5 -> CSMA/CA MAC Layer/5(SigD)  "<signal5>"
  TxLength/1 -> Bus Creator/1
  TxEn/1 -> Bus Creator/2
  Bus Selector1/6 -> CSMA/CA MAC Layer/6(RxErr)  "<signal6>"
  RxDataOk/1 -> Bus Creator/3
  BusSwitchFunOut/1(Out1) -> Bus Selector3/1
  MAC_Sel/1 -> BusSwitchFunIn/1(Sel), BusSwitchFunOut/1(Sel)
  SigDet/1 -> Bus Creator/5
  CSMA/CA MAC Layer/4(TxAckOn) -> Bus Creator2/4
  CSMA/CA MAC Layer/2(TxDataDone) -> Bus Creator2/2
  BusSwitchFunIn/1(Out) -> Bus Selector2/1
  Bus Creator2/1 -> BusSwitchFunIn/3(In2)
  ALOHA MAC Layer/5(BOTime) -> Bus Creator1/5
  CSMA/CA MAC Layer/5(BOTime) -> Bus Creator2/5
  CSMA/CA MAC Layer/6(AckWaitTime) -> Bus Creator2/6
  ALOHA MAC Layer/4(TxAckOn) -> Bus Creator1/4
  ALOHA MAC Layer/2(TxDataDone) -> Bus Creator1/2
  ALOHA MAC Layer/3(TxDataOn) -> Bus Creator1/3
  ALOHA MAC Layer/1(TxDataFail) -> Bus Creator1/1
  Bus Selector2/1 -> TXDataFail/1  "<signal1>"
  Bus Selector2/2 -> TxDataDone/1  "<signal2>"
  Bus Selector2/6 -> Terminator3/1  "<signal6>"
  Bus Selector2/5 -> BoTime/1  "<signal5>"
  Bus Selector2/3 -> TXDataOn/1  "<signal3>"
  ALOHA MAC Layer/6(AckWaitTime) -> Bus Creator1/6
  Bus Creator1/1 -> BusSwitchFunIn/2(In1)
  CSMA/CA MAC Layer/1(TxDataFail) -> Bus Creator2/1
  Bus Selector2/4 -> TxAckOn/1  "<signal4>"
  CSMA/CA MAC Layer/3(TxDataOn) -> Bus Creator2/3
  Bus Selector3/5 -> Terminator/1  "<signal5>"
  Bus Selector3/6 -> Terminator1/1  "<signal6>"
  CSMA/CA MAC Layer/7(Retry) -> Terminator2/1

== system PacketizedNetworkLib/PHY//MAC Transceiver/Tx//RxSwitch&Flts3 ==
  Tx_in : Inport
  Rx_in : Inport  Port=2
  Control1 : Inport  Port=3
  Constant : Constant  Value=complex(0)  SampleTime=Ts/2
  Constant1 : Constant  Value=complex(0)
  Downsample : DownSample  RateOptions=Allow multirate processing
  Not 1 : Logic  Operator=NOT  AllPortsSameDT=off  OutDataTypeStr=boolean
  Raised Cosine Receive HDL Filter3 : commfilt2/Raised Cosine Receive Filter  filtType=Square root  R=0.2  filtSpan=10  N=6  downFactor=3  downOffset=0  filterGain=1  RateOptions=Allow multirate processing  framing=Mute  checkCoeff=off  variableName=rcRxFilt3  currentFiltSpan=10  D=5  inputOffset=0  sampMode=Mute  saveAsFlag=0  rateMode=Downsampling  checkGain=Normalized  launchFVT=on  roundingMode=Floor  overflowMode=off  coeffDataTypeStr=Inherit: Same word length as input  coeffMin=[]  coeffMax=[]  coeffLastDataTypeStr=Inherit: Same word length as input  accumDataTypeStr=Inherit: Same as product output  accumLastDataTypeStr=Inherit: Same as product output  outputDataTypeStr=Inherit: Same as accumulator  outputMin=[]  outputMax=[]  outputLastDataTypeStr=Inherit: Same as accumulator
  Raised Cosine Transmit HDL Filter : commfilt2/Raised Cosine Transmit Filter  filtType=Square root  R=0.2  filtSpan=10  N=6  filterGain=1  RateOptions=Allow multirate processing  framing=Mute  checkCoeff=off  variableName=rcTxFilt  checkGain=Normalized  sampMode=Mute  saveAsFlag=0  currentFiltSpan=10  D=5  launchFVT=on  roundingMode=Floor  overflowMode=off  coeffDataTypeStr=Inherit: Same word length as input  coeffMin=[]  coeffMax=[]  coeffLastDataTypeStr=Inherit: Same word length as input  outputDataTypeStr=Inherit: Same as accumulator  outputMin=[]  outputMax=[]  outputLastDataTypeStr=Inherit: Same as accumulator
  Switch2 : Switch  Criteria=u2 > Threshold  SaturateOnIntegerOverflow=off  InputSameDT=off
  Switch3 : Switch  Criteria=u2 > Threshold  SaturateOnIntegerOverflow=off  InputSameDT=off
  Tx_out : Outport  VectorParamsAs1DForOutWhenUnconnected=off
  Rx_out : Outport  Port=2  VectorParamsAs1DForOutWhenUnconnected=off
  wires:
  Tx_in/1 -> Switch2/1
  Switch3/1 -> Rx_out/1
  Raised Cosine Receive HDL Filter3/1 -> Switch3/1
  Constant/1 -> Switch3/3
  Constant1/1 -> Switch2/3
  Control1/1 -> Downsample/1, Not 1/1
  Rx_in/1 -> Raised Cosine Receive HDL Filter3/1
  Switch2/1 -> Raised Cosine Transmit HDL Filter/1
  Raised Cosine Transmit HDL Filter/1 -> Tx_out/1
  Not 1/1 -> Switch3/2
  Downsample/1 -> Switch2/2

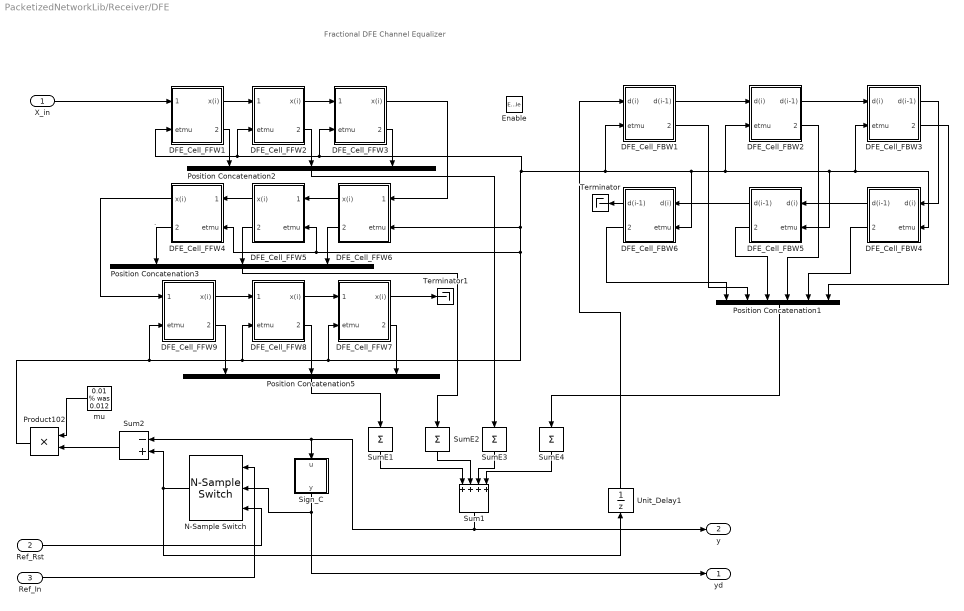
== system PacketizedNetworkLib/Receiver/DFE  ==
  note: .
  note: Fractional DFE Channel Equalizer
  X_in : Inport
  "Ref_Rst " : Inport  Port=2
  Ref_In : Inport  Port=3
  Enable : EnablePort
  DFE_Cell_FBW1 : Subsystem
  DFE_Cell_FBW2 : Subsystem
  DFE_Cell_FBW3 : Subsystem
  DFE_Cell_FBW4 : Subsystem
  DFE_Cell_FBW5 : Subsystem
  DFE_Cell_FBW6 : Subsystem
  DFE_Cell_FFW1 : Subsystem
  DFE_Cell_FFW2 : Subsystem
  DFE_Cell_FFW3 : Subsystem
  DFE_Cell_FFW4 : Subsystem
  DFE_Cell_FFW5 : Subsystem
  DFE_Cell_FFW6 : Subsystem
  DFE_Cell_FFW7 : Subsystem
  DFE_Cell_FFW8 : Subsystem
  DFE_Cell_FFW9 : Subsystem
  N-Sample Switch : dspswit3/N-Sample Switch  N=152  reset=on  TriggerType=Rising edge  Ts=-1
  Position Concatenation1 : Concatenate  NumInputs=6  ConcatenateDimension=6
  Position Concatenation2 : Concatenate  NumInputs=3  ConcatenateDimension=3
  Position Concatenation3 : Concatenate  NumInputs=3  ConcatenateDimension=3
  Position Concatenation5 : Concatenate  NumInputs=3  ConcatenateDimension=3
  Product102 : Product  InputSameDT=on  RndMeth=Zero  SaturateOnIntegerOverflow=on  OutDataTypeStr=Inherit: Same as first input
  "Sign_C " : MATLAB Function  TreatAsAtomicUnit=on
  Sum1 : Sum  Inputs=++++  InputSameDT=on  SaturateOnIntegerOverflow=on  OutDataTypeStr=Inherit: Same as first input
  Sum2 : Sum  Inputs=-+  InputSameDT=on  SaturateOnIntegerOverflow=on  OutDataTypeStr=Inherit: Same as first input
  SumE{1..4} (4 alike) : Sum  Inputs=+
  Terminator : Terminator
  Terminator1 : Terminator
  "Unit_Delay1 " : UnitDelay  SampleTime=-1  HasFrameUpgradeWarning=on
  mu : Constant  Value="0.01  % was 0.012"  SampleTime=-1
  yd : Outport  VectorParamsAs1DForOutWhenUnconnected=off
  y : Outport  Port=2  VectorParamsAs1DForOutWhenUnconnected=off
  wires:
  DFE_Cell_FFW5/1("x(i) ") -> DFE_Cell_FFW4/1(x(i+1))
  DFE_Cell_FFW6/2(y(i+1)) -> Position Concatenation3/3
  Position Concatenation2/1 -> SumE3/1
  Position Concatenation3/1 -> SumE2/1
  DFE_Cell_FBW4/1("d(i-1) ") -> DFE_Cell_FBW5/1(d(i))
  DFE_Cell_FFW8/2(y(i+1)) -> Position Concatenation5/2
  DFE_Cell_FBW1/1("d(i-1) ") -> DFE_Cell_FBW2/1(d(i))
  DFE_Cell_FFW4/2(y(i+1)) -> Position Concatenation3/1
  "Unit_Delay1 "/1 -> DFE_Cell_FBW1/1(d(i))
  DFE_Cell_FFW9/2(y(i+1)) -> Position Concatenation5/1
  "Sign_C "/1(y) -> yd/1, N-Sample Switch/2
  DFE_Cell_FFW7/2(y(i+1)) -> Position Concatenation5/3
  SumE2/1 -> Sum1/2
  DFE_Cell_FFW3/2(y(i+1)) -> Position Concatenation2/3
  DFE_Cell_FFW7/1("x(i) ") -> Terminator1/1
  DFE_Cell_FFW4/1("x(i) ") -> DFE_Cell_FFW9/1(x(i+1))
  Sum1/1 -> y/1, "Sign_C "/1(u), Sum2/1
  DFE_Cell_FFW2/2(y(i+1)) -> Position Concatenation2/2
  DFE_Cell_FBW1/2(yd(i+1)) -> Position Concatenation1/2
  DFE_Cell_FFW1/2(y(i+1)) -> Position Concatenation2/1
  SumE1/1 -> Sum1/1
  DFE_Cell_FFW6/1("x(i) ") -> DFE_Cell_FFW5/1(x(i+1))
  DFE_Cell_FFW5/2(y(i+1)) -> Position Concatenation3/2
  DFE_Cell_FBW6/1("d(i-1) ") -> Terminator/1
  Sum2/1 -> Product102/2
  DFE_Cell_FBW3/1("d(i-1) ") -> DFE_Cell_FBW4/1(d(i))
  Product102/1 -> DFE_Cell_FFW9/2(etmu), DFE_Cell_FFW8/2(etmu), DFE_Cell_FFW7/2(etmu), DFE_Cell_FFW5/2(etmu), DFE_Cell_FFW4/2(etmu), DFE_Cell_FFW6/2(etmu), DFE_Cell_FFW1/2(etmu), DFE_Cell_FFW2/2(etmu), DFE_Cell_FFW3/2(etmu), DFE_Cell_FBW1/2(etmu), DFE_Cell_FBW6/2(etmu), DFE_Cell_FBW2/2(etmu), DFE_Cell_FBW5/2(etmu), DFE_Cell_FBW4/2(etmu), DFE_Cell_FBW3/2(etmu)
  SumE3/1 -> Sum1/3
  mu/1 -> Product102/1
  N-Sample Switch/1 -> "Unit_Delay1 "/1, Sum2/2
  Position Concatenation1/1 -> SumE4/1
  DFE_Cell_FFW3/1("x(i) ") -> DFE_Cell_FFW6/1(x(i+1))
  DFE_Cell_FFW2/1("x(i) ") -> DFE_Cell_FFW3/1(x(i+1))
  DFE_Cell_FBW2/2(yd(i+1)) -> Position Concatenation1/4
  DFE_Cell_FBW4/2(yd(i+1)) -> Position Concatenation1/5
  DFE_Cell_FBW5/2(yd(i+1)) -> Position Concatenation1/3
  DFE_Cell_FBW5/1("d(i-1) ") -> DFE_Cell_FBW6/1(d(i))
  DFE_Cell_FBW6/2(yd(i+1)) -> Position Concatenation1/1
  DFE_Cell_FBW2/1("d(i-1) ") -> DFE_Cell_FBW3/1(d(i))
  SumE4/1 -> Sum1/4
  DFE_Cell_FFW1/1("x(i) ") -> DFE_Cell_FFW2/1(x(i+1))
  Position Concatenation5/1 -> SumE1/1
  DFE_Cell_FBW3/2(yd(i+1)) -> Position Concatenation1/6
  DFE_Cell_FFW9/1("x(i) ") -> DFE_Cell_FFW8/1(x(i+1))
  DFE_Cell_FFW8/1("x(i) ") -> DFE_Cell_FFW7/1(x(i+1))
  Ref_In/1 -> N-Sample Switch/1
  X_in/1 -> DFE_Cell_FFW1/1(x(i+1))
  "Ref_Rst "/1 -> N-Sample Switch/3

== system PacketizedNetworkLib/Receiver/REF_LUT ==
  En : Inport
  1-D Lookup Table1 : Lookup_n-D  NumberOfTableDimensions=1  LookupTableObject=''  BreakpointsSpecification=Even spacing  BreakpointsForDimension1=[-5:5]  BreakpointsForDimension2FirstPoint=10  BreakpointsForDimension2Spacing=12  BreakpointsForDimension1DataTypeStr=int16  IndexSearchMethod=Evenly spaced points  Table=dfeRef  TableDataTypeStr=double  InterpMethod=Flat  DiagnosticForOutOfRangeInput=Error  InternalRulePriority=Speed  OutDataTypeStr=double  RndMeth=Simplest
  Data Type Conversion2 : DataTypeConversion  OutDataTypeStr=boolean  SaturateOnIntegerOverflow=off  RndMeth=Floor
  Data Type Conversion3 : DataTypeConversion  OutDataTypeStr=boolean  SaturateOnIntegerOverflow=off  RndMeth=Floor
  HDL Counter3 : hdlsllib/Sources/HDL Counter  CountType=Count limited  CountInit=1  CountStep=1  CountMax=160  CountFromType=Initial value  CountFrom=1  CountResetPort=on  CountLoadPort=off  CountEnbPort=on  CountDirPort=off  CountHitOutputPort=off  CountDataType=Unsigned  CountWordLen=8  CountFracLen=0  CountSampTime=1
  N-Sample Enable : dspswit3/N-Sample Enable  N=160  ActiveLevel=High (1)  reset=on  TriggerType=Either edge  Ts=-1  DataType=Logical
  DataOut : Outport  VectorParamsAs1DForOutWhenUnconnected=off
  wires:
  Data Type Conversion2/1 -> HDL Counter3/1
  Data Type Conversion3/1 -> HDL Counter3/2
  HDL Counter3/1 -> 1-D Lookup Table1/1
  1-D Lookup Table1/1 -> DataOut/1
  En/1 -> N-Sample Enable/1, Data Type Conversion3/1
  N-Sample Enable/1 -> Data Type Conversion2/1

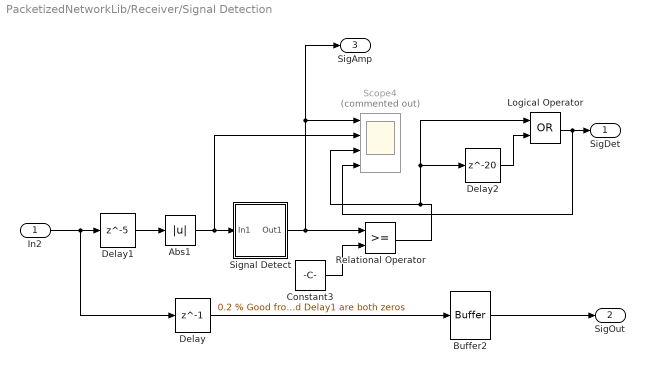
== system PacketizedNetworkLib/Receiver/Signal Detection ==
  In2 : Inport
  Abs1 : Abs  SaturateOnIntegerOverflow=off
  Buffer2 : Buffer  N=2  OutputFrames=off
  Constant3 : Constant  Value=0.2 % Good from 1.3 to 0.3 at Delay and Delay1 are both zeros  OutDataTypeStr=double  SampleTime=-1
  Delay : Delay  DelayLength=1
  Delay1 : Delay  DelayLength=5
  Delay2 : Delay  DelayLength=20
  Logical Operator : Logic  Operator=OR  AllPortsSameDT=off  OutDataTypeStr=boolean
  Relational Operator : RelationalOperator  OutDataTypeStr=boolean  RndMeth=Simplest  InputSameDT=off
  Scope4 : Scope  Commented=on  NumInputPorts=4
      settings: ActiveDisplayYMinimum=-0.4844  ActiveDisplayYMaximum=4.35956
  Signal Detect : Subsystem
  SigDet : Outport  VectorParamsAs1DForOutWhenUnconnected=off
  SigOut : Outport  Port=2  VectorParamsAs1DForOutWhenUnconnected=off
  SigAmp : Outport  Port=3  VectorParamsAs1DForOutWhenUnconnected=off
  wires:
  Buffer2/1 -> SigOut/1
  Delay/1 -> Buffer2/1
  Signal Detect/1(Out1) -> Relational Operator/1, Scope4/1, SigAmp/1
  Abs1/1 -> Scope4/2, Signal Detect/1(In1)
  Constant3/1 -> Relational Operator/2
  Relational Operator/1 -> Delay2/1, Logical Operator/1, Scope4/3
  Delay1/1 -> Abs1/1
  In2/1 -> Delay1/1, Delay/1
  Logical Operator/1 -> Scope4/4, SigDet/1
  Delay2/1 -> Logical Operator/2

== system PacketizedNetworkLib/Transmitter/PlsDly1 ==
  In : Inport
  Delay2 : Delay  DelayLength=32
  Logical Operator : Logic  Operator=OR  AllPortsSameDT=off  OutDataTypeStr=boolean
  Out : Outport  VectorParamsAs1DForOutWhenUnconnected=off
  wires:
  Logical Operator/1 -> Out/1
  In/1 -> Delay2/1, Logical Operator/1
  Delay2/1 -> Logical Operator/2

== system PacketizedNetworkLib/Transmitter/TxAck_LUT ==
  En : Inport
  Ack : Inport  Port=2
  Data Type Conversion3 : DataTypeConversion  OutDataTypeStr=boolean  SaturateOnIntegerOverflow=off  RndMeth=Floor
  HDL Counter3 : hdlsllib/Sources/HDL Counter  CountType=Count limited  CountInit=1  CountStep=1  CountMax=AckLength  CountFromType=Initial value  CountFrom=1  CountResetPort=on  CountLoadPort=off  CountEnbPort=on  CountDirPort=off  CountHitOutputPort=off  CountDataType=Unsigned  CountWordLen=16  CountFracLen=0  CountSampTime=1
  Logical Operator : Logic  Operator=NOT  AllPortsSameDT=off  OutDataTypeStr=boolean
  Signal Specification : SignalSpecification  Dimensions=1
  Variable Selector : dspindex/Variable Selector  NumInputs=1  rowsOrCols=Rows  IdxMode=Variable  Elements=[1 3]  ZerOneIdxMode=One-based  errmode=Clip Index  FillMode=on  FillValues=0
  DataOut : Outport  VectorParamsAs1DForOutWhenUnconnected=off
  wires:
  En/1 -> Logical Operator/1, Data Type Conversion3/1
  Variable Selector/1 -> DataOut/1
  HDL Counter3/1 -> Signal Specification/1
  Data Type Conversion3/1 -> HDL Counter3/2
  Logical Operator/1 -> HDL Counter3/1
  Signal Specification/1 -> Variable Selector/2
  Ack/1 -> Variable Selector/1

== system PacketizedNetworkLib/Transmitter/TxData_LUT ==
  En : Inport
  Data : Inport  Port=2
  Data Type Conversion3 : DataTypeConversion  OutDataTypeStr=boolean  SaturateOnIntegerOverflow=off  RndMeth=Floor
  HDL Counter3 : hdlsllib/Sources/HDL Counter  CountType=Count limited  CountInit=1  CountStep=1  CountMax=DataLength  CountFromType=Initial value  CountFrom=1  CountResetPort=on  CountLoadPort=off  CountEnbPort=on  CountDirPort=off  CountHitOutputPort=off  CountDataType=Unsigned  CountWordLen=16  CountFracLen=0  CountSampTime=1
  Logical Operator : Logic  Operator=NOT  AllPortsSameDT=off  OutDataTypeStr=boolean
  Signal Specification : SignalSpecification  Dimensions=1
  Variable Selector : dspindex/Variable Selector  NumInputs=1  rowsOrCols=Rows  IdxMode=Variable  Elements=[1 3]  ZerOneIdxMode=One-based  errmode=Clip Index  FillMode=on  FillValues=0
  DataOut : Outport  VectorParamsAs1DForOutWhenUnconnected=off
  wires:
  En/1 -> Logical Operator/1, Data Type Conversion3/1
  HDL Counter3/1 -> Signal Specification/1
  Data Type Conversion3/1 -> HDL Counter3/2
  Logical Operator/1 -> HDL Counter3/1
  Signal Specification/1 -> Variable Selector/2
  Data/1 -> Variable Selector/1
  Variable Selector/1 -> DataOut/1
